simulink model "rlMpptModel"  (R2022a)
settings: Solver=ode23tb  StartTime=0.0  StopTime=0.5  FixedStep=Ts  RelTol=1e-4
model workspace (MAT data in the model file):
  Ir1 = 900
  Ir2 = 300
  Ir3 = 250
  PMmpStc = 1005
  Pmmtstc = 1004.715
  T1 = 25
  T2 = 25
  T3 = 25
  initialDuty = 0.5
libraries: spsDiodeLib x4, simulink x4, spsSeriesRLCBranchLib x4, spsPVArrayLib x3, spsCurrentMeasurementLib x1, spsIGBTDiodeLib x1, spsPWMGeneratorDCDCLib x1, spsVoltageMeasurementLib x1, rllib x1, spspowerguiLib x1
settings Model: SimulationMode=accelerator  Creator=MathWorks  LastModifiedBy=archi
settings SolverCC: AlgebraicLoopSolver=LineSearch  SolverResetMethod=Robust
settings DataIOCC: LimitDataPoints=on  SaveFormat=Array  SignalLoggingSaveFormat=ModelDataLogs
settings OptimizationCC: ExpressionDepthLimit=2147483647  LifeSpan=inf
settings DebuggingCC: UnderspecifiedInitializationDetection=Classic  MergeDetectMultiDrivingBlocksExec=none  SolverPrmCheckMsg=warning  UnconnectedInputMsg=warning  UnconnectedOutputMsg=warning  UnconnectedLineMsg=warning  AllowSymbolicDim=off  StateNameClashWarn=warning  SFUnexpectedBacktrackingDiag=warning  SFNoUnconditionalDefaultTransitionDiag=warning  SFExecutionAtInitializationDiag=none  SFMachineParentedDataDiag=warning  ArithmeticOperatorsInVariantConditions=warning
settings HardwareCC: ProdBitPerPointer=32  ProdBitPerSizeT=32  ProdBitPerPtrDiffT=32  ProdLargestAtomicFloat=None  ProdIntDivRoundTo=Undefined  ProdEndianess=Unspecified  ProdWordSize=32  ProdHWDeviceType=32-bit Generic
settings ModelReferenceCC: PropagateSignalLabelsOutOfModel=off
settings SFSimCC: SimUseLocalCustomCode=off  CustomCodeUndefinedFunction=UseInterfaceOnly
settings RTWCC: RTWUseLocalCustomCode=off
settings CodeAppCC: StateflowObjectComments=on
settings GRTTargetCC: TargetLangStandard=C89/C90 (ANSI)  CombineOutputUpdateFcns=off  GRTInterface=on
settings ConfigComp: CovMetricSettings=dw  CovSaveCumulativeToWorkspaceVar=on  CovSaveSingleToWorkspaceVar=on  CovExternalEMLEnable=off  CovSFcnEnable=off
settings SimscapeCC: SimscapeNormalizeSystem=off

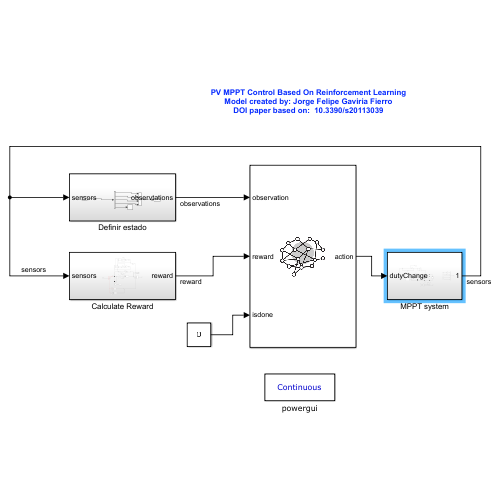
[thumbnail: Simulink's stored preview of the top-level diagram]
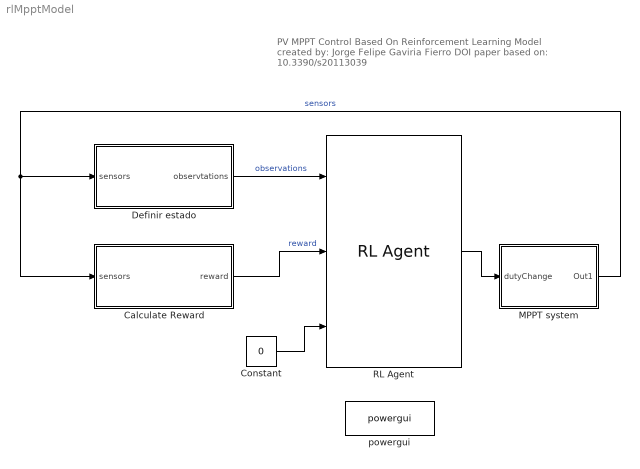
== system rlMpptModel ==
  note: PV MPPT Control Based On Reinforcement Learning
      | Model created by: Jorge Felipe Gaviria Fierro
      | DOI paper based on: 10.3390/s20113039
  Calculate Reward : Subsystem
  Constant : Constant  Value=0
  Definir estado : Subsystem
  MPPT system : Subsystem
  RL Agent : rllib/RL Agent  Agent=agentObj  ExternalActionAsInput=off  ProvideLastAction=off  ProvideCumRwd=off  TreatAsDirectFeedthrough=on  UseStrictObservationDataTypes=off
  powergui : spspowerguiLib/powergui  Priority=1  SimulationMode=Continuous  SampleTime=0.00001  frequency=60  Iterations=50  frequencyindice=0  Pbase=100e6  ErrMax=1e-4  UnitsV=kV  UnitsW=MW  buscounter=0  FunctionMessages=off  echomessages=off  EnableUseOfTLC=off  CurrentSourceSwitches=on  DisableSnubberDevices=on  DisableRonSwitches=off  DisableVfSwitches=off  DisplayEquations=off  AutomaticDiscreteSolvers=off  SolverType=Tustin/Backward Euler (TBE)  Interpol=off  ExternalGateDelay=off  methode=off  Ts=0  x0status=blocks  SPID=off  SwTol=0  HookPort=off  NonlinearTolerance=1e-4  nMaxIteration=100  ContinueOnMaxIteration=off  RestoreLinks=warning  ResistiveCurrentMeasurement=off  Frange=[0:2:500]  Ylog=off  Xlog=on  ShowGrid=off  save=off  variable=ZData  structure=0  ZoomFFT=on  StartTime=0.0  cycles=1  DisplayStyle=1  fundamental=60  FreqAxis=off  MaxFrequency=1000  frequencyindicesteady=1  RmsSteady=1  display=off
  wires:
  RL Agent/1 -> MPPT system/1(dutyChange)
  MPPT system/1(Out1) -> Calculate Reward/1(sensors), Definir estado/1(sensors)  "sensors"
  Definir estado/1(observtations) -> RL Agent/1  "observations"
  Constant/1 -> RL Agent/3
  Calculate Reward/1(reward) -> RL Agent/2  "reward"

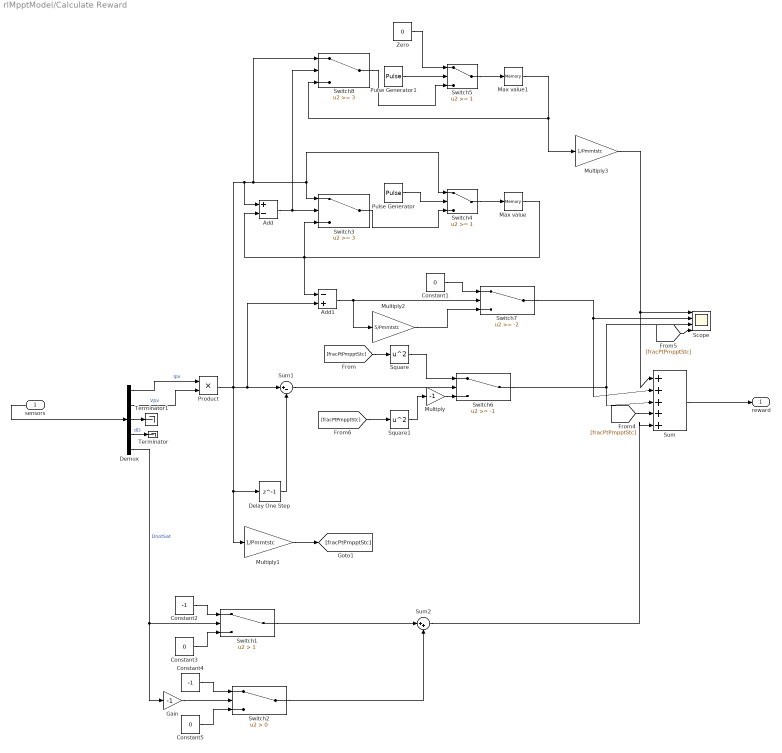
== system rlMpptModel/Calculate Reward ==
  sensors : Inport
  Add : Sum  Inputs=+-
  Add1 : Sum  Inputs=-+
  Constant1 : Constant  Value=0
  Constant2 : Constant  Value=-1
  Constant3 : Constant  Value=0
  Constant4 : Constant  Value=-1
  Constant5 : Constant  Value=0
  Delay One Step : Delay  DelayLength=1  SampleTime=0.01
  Demux : Demux  Outputs=5
  Gain : Gain  Gain=-1
  Max value : Memory
  Max value1 : Memory
  Multiply : Gain  Gain=-1
  Multiply1 : Gain  Gain=1/Pmmtstc
  Multiply2 : Gain  Gain=5/Pmmtstc
  Multiply3 : Gain  Gain=1/Pmmtstc
  Product : Product
  Pulse Generator : DiscretePulseGenerator  PulseType=Time based  Period=0.504
  Pulse Generator1 : DiscretePulseGenerator  PulseType=Time based  Period=0.0105
  Scope : Scope  NumInputPorts=4
  Square : Math  Operator=square
  Square1 : Math  Operator=square
  Sum : Sum  Inputs=|+++++
  Sum1 : Sum  Inputs=|+-
  Sum2 : Sum  Inputs=|++
  Switch1 : Switch  Criteria=u2 > Threshold  Threshold=1  SaturateOnIntegerOverflow=off  InputSameDT=off
  Switch2 : Switch  Criteria=u2 > Threshold  SaturateOnIntegerOverflow=off  InputSameDT=off
  Switch3 : Switch  Threshold=3  SaturateOnIntegerOverflow=off  InputSameDT=off
  Switch4 : Switch  Threshold=1  SaturateOnIntegerOverflow=off  InputSameDT=off
  Switch5 : Switch  Threshold=1  SaturateOnIntegerOverflow=off  InputSameDT=off
  Switch6 : Switch  Threshold=-1  SaturateOnIntegerOverflow=off  InputSameDT=off
  Switch7 : Switch  Threshold=-2  SaturateOnIntegerOverflow=off  InputSameDT=off
  Switch8 : Switch  Threshold=3  SaturateOnIntegerOverflow=off  InputSameDT=off
  Terminator : Terminator
  Terminator1 : Terminator
  Zero : Constant  Value=0  OutDataTypeStr=Inherit: Inherit via back propagation
  reward : Outport
  wires:
  sensors/1 -> Demux/1
  Demux/1 -> Product/1  "Ipv"
  Demux/2 -> Product/2  "Vpv"
  Sum/1 -> reward/1
  Delay One Step/1 -> Sum1/2
  Constant2/1 -> Switch1/1
  Constant3/1 -> Switch1/3
  Switch1/1 -> Sum2/1
  Constant5/1 -> Switch2/3
  Constant4/1 -> Switch2/1
  Gain/1 -> Switch2/2
  Switch2/1 -> Sum2/2
  Demux/4 -> Terminator/1  "dD"
  Demux/3 -> Terminator1/1
  Sum2/1 -> Sum/5
  Demux/5 -> Switch1/2, Gain/1  "DnotSat"
  Max value/1 -> Add1/1, Switch3/3, Add/2
  Pulse Generator/1 -> Switch4/2
  Product/1 -> Multiply1/1, Delay One Step/1, Sum1/1, Add1/2, Add/1, Switch8/1, Switch3/1, Switch4/1
  Switch4/1 -> Max value/1
  Switch7/1 -> Sum/2, Scope/2
  Add/1 -> Switch8/2, Switch3/2
  Sum1/1 -> Switch6/2
  Square/1 -> Switch6/1
  Square1/1 -> Multiply/1
  Switch6/1 -> Sum/3, Scope/3
  Multiply3/1 -> Scope/1, Sum/1
  Add1/1 -> Multiply2/1, Switch7/2
  Constant1/1 -> Switch7/1
  Switch5/1 -> Max value1/1
  Switch3/1 -> Switch4/3
  Pulse Generator1/1 -> Switch5/2
  Max value1/1 -> Multiply3/1, Switch8/3
  Switch8/1 -> Switch5/3
  Zero/1 -> Switch5/1
  Multiply1/1 -> [fracPtPmpptStc]
  [fracPtPmpptStc] -> Square/1
  [fracPtPmpptStc] -> Sum/4
  [fracPtPmpptStc] -> Scope/4
  [fracPtPmpptStc] -> Square1/1
  Multiply2/1 -> Switch7/3
  Multiply/1 -> Switch6/3

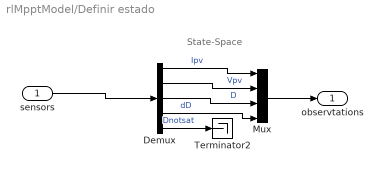
== system rlMpptModel/Definir estado ==
  note: State-Space
  sensors : Inport
  Demux : Demux  Outputs=5
  Mux : Mux
  Terminator2 : Terminator
  observtations : Outport
  wires:
  Demux/4 -> Mux/4  "dD"
  Demux/1 -> Mux/1  "Ipv"
  Demux/2 -> Mux/2  "Vpv"
  sensors/1 -> Demux/1
  Mux/1 -> observtations/1
  Demux/3 -> Mux/3  "D"
  Demux/5 -> Terminator2/1  "Dnotsat"

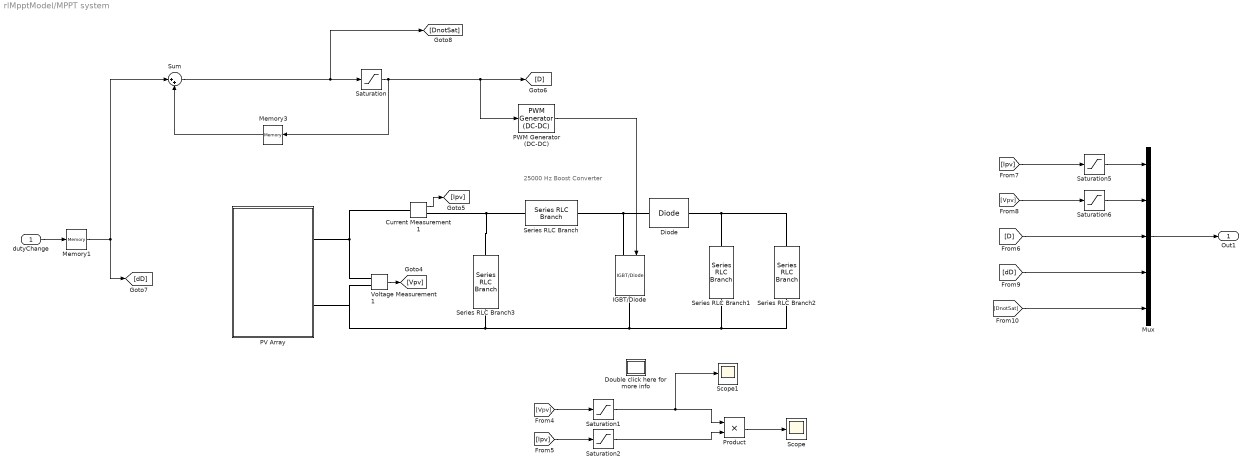
== system rlMpptModel/MPPT system ==
  note: 25000 Hz
      | Boost Converter
  dutyChange : Inport
  Current Measurement1 : spsCurrentMeasurementLib/Current Measurement  PhasorSimulation=off  OutputType=Complex  PSBequivalent=0
  Diode : spsDiodeLib/Diode  Ron=0.001  Lon=0  Vf=0.8  IC=0  UseSnubber=0  Rs=500  Cs=inf  Measurements=off
  Double click here for more info : Subsystem
      settings: OpenFcn=showdemo(bdroot(gcb))
      mask Display: disp('?')
  IGBT/Diode : spsIGBTDiodeLib/IGBT//Diode  Ron=1e-3  Rs=1e5  Cs=inf  Measurements=off
  Memory1 : Memory  InheritSampleTime=on
  Memory3 : Memory  InitialCondition=initialDuty  InheritSampleTime=on
  Mux : Mux  Inputs=5
  PV Array : Subsystem
  PWM Generator (DC-DC) : spsPWMGeneratorDCDCLib/PWM Generator (DC-DC)  Fsw=25000  Ts=0
  Product : Product
  Saturation : Saturate  UpperLimit=1  LowerLimit=0
  Saturation1 : Saturate  UpperLimit=1000000000000000  LowerLimit=0
  Saturation2 : Saturate  UpperLimit=1000000000000000000  LowerLimit=0
  Saturation5 : Saturate  UpperLimit=1000000000000  LowerLimit=0
  Saturation6 : Saturate  UpperLimit=10000000000000000  LowerLimit=0
  Scope : Scope
  Scope1 : Scope
  Series RLC Branch : spsSeriesRLCBranchLib/Series RLC Branch  LConnTagsString=__new0  RConnTagsString=__new0  BranchType=L  Resistance=1  Inductance=2.057e-3  SetiL0=off  InitialCurrent=0  Capacitance=1e-6  Setx0=off  InitialVoltage=0  Measurements=None
  Series RLC Branch1 : spsSeriesRLCBranchLib/Series RLC Branch  LConnTagsString=__new0  RConnTagsString=__new0  BranchType=C  Resistance=1  Inductance=1e-3  SetiL0=off  InitialCurrent=0  Capacitance=1.29e-05  Setx0=off  InitialVoltage=0  Measurements=None
  Series RLC Branch2 : spsSeriesRLCBranchLib/Series RLC Branch  LConnTagsString=__new0  RConnTagsString=__new0  BranchType=R  Resistance=61.71003717  Inductance=1e-3  SetiL0=off  InitialCurrent=0  Capacitance=1e-6  Setx0=off  InitialVoltage=0  Measurements=None
  Series RLC Branch3 : spsSeriesRLCBranchLib/Series RLC Branch  LConnTagsString=__new0  RConnTagsString=__new0  BranchType=C  Resistance=1e-4  Inductance=1.032e-3  SetiL0=off  InitialCurrent=0  Capacitance=3e-3  Setx0=off  InitialVoltage=0  Measurements=None
  Sum : Sum  Inputs=|++
  Voltage Measurement1 : spsVoltageMeasurementLib/Voltage Measurement  PhasorSimulation=off  OutputType=Complex  PSBequivalent=0
  Out1 : Outport
  wires:
  dutyChange/1 -> Memory1/1
  [Vpv] -> Saturation1/1
  Current Measurement1/1 -> [Ipv]
  [Ipv] -> Saturation2/1
  Voltage Measurement1/1 -> [Vpv]
  Mux/1 -> Out1/1
  PWM Generator (DC-DC)/1 -> IGBT/Diode/1
  [DnotSat] -> Mux/5
  [dD] -> Mux/4
  [D] -> Mux/3
  Memory1/1 -> Sum/1, [dD]
  Memory3/1 -> Sum/2
  Saturation1/1 -> Scope1/1, Product/1
  Saturation2/1 -> Product/2
  [Ipv] -> Saturation5/1
  [Vpv] -> Saturation6/1
  Saturation5/1 -> Mux/1
  Saturation6/1 -> Mux/2
  Sum/1 -> [DnotSat], Saturation/1
  Saturation/1 -> PWM Generator (DC-DC)/1, [D], Memory3/1
  Product/1 -> Scope/1
  connections:
  Series RLC Branch2/RConn1 -- Series RLC Branch1/RConn1 -- Voltage Measurement1/LConn2 -- PV Array/RConn2 -- Series RLC Branch3/RConn1 -- IGBT/Diode/RConn1
  Series RLC Branch3/LConn1 -- Current Measurement1/RConn1 -- Series RLC Branch/LConn1
  PV Array/RConn1 -- Voltage Measurement1/LConn1 -- Current Measurement1/LConn1
  Diode/RConn1 -- Series RLC Branch1/LConn1 -- Series RLC Branch2/LConn1
  Diode/LConn1 -- IGBT/Diode/LConn1 -- Series RLC Branch/RConn1

== system rlMpptModel/MPPT system/Double click here for more info ==

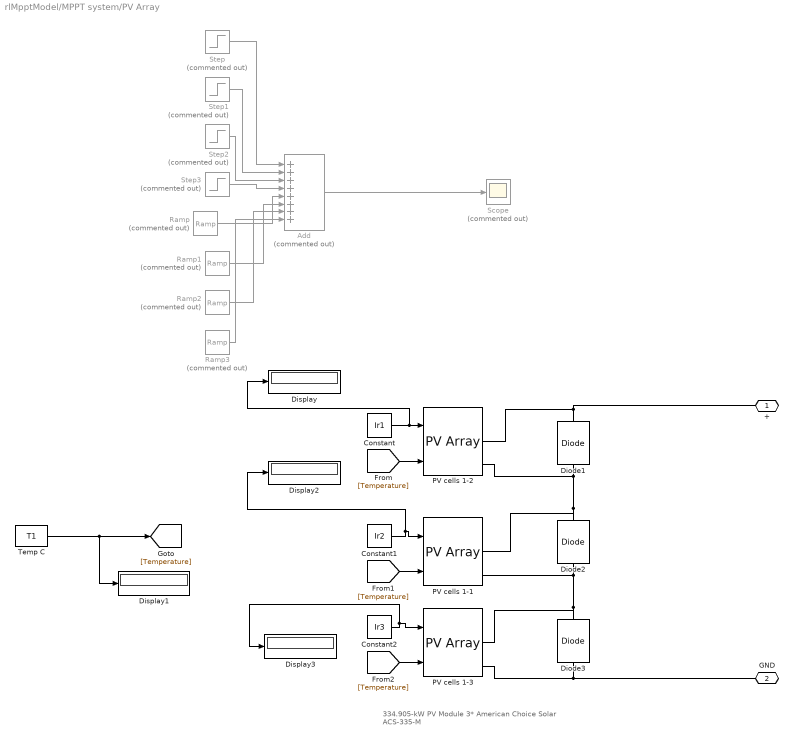
== system rlMpptModel/MPPT system/PV Array ==
  note: 334.905-kW  PV Module
      | 3* American Choice Solar ACS-335-M
  Add : Sum  Commented=on  Inputs=++++++++
  Constant : Constant  Value=Ir1
  Constant1 : Constant  Value=Ir2
  Constant2 : Constant  Value=Ir3
  Diode1 : spsDiodeLib/Diode  Ron=0.001  Lon=0  Vf=0.7  IC=0  UseSnubber=off  Rs=1e5*inf  Cs=inf  Measurements=off
  Diode2 : spsDiodeLib/Diode  Ron=0.001  Lon=0  Vf=0.7  IC=0  UseSnubber=off  Rs=1e5*inf  Cs=inf  Measurements=off
  Diode3 : spsDiodeLib/Diode  Ron=0.001  Lon=0  Vf=0.7  IC=0  UseSnubber=off  Rs=1e5*inf  Cs=inf  Measurements=off
  Display{,1..3} (4 alike) : Display
  PV cells 1-1 : spsPVArrayLib/PV Array  Npar=1  Nser=1  PlotType=array @ 25 deg.C & specified irradiances  S_vec="[ 1000  500  100 ]"  Temp_C_vec="[ 45 25  ]"  ModuleName=User-defined  PlotWhenSelected=off  Pm=334.905  Ncell=80  Voc=49.9  Isc=9  Vm=41.5  Im=8.07  beta_Voc_pc=-0.36  alpha_Isc_pc=0.09  beta_Voc=-0.17964  alpha_Isc=0.0081  IL=9.0297  I0=3.1312e-10  nI=1.0111  Rsh=77.6407  Rs=0.25633  RobustModel=off  RobustCellTemperature=25  BAL=on  Tc=1e-5  Tfilter=5e-5
  PV cells 1-2 : spsPVArrayLib/PV Array  Npar=1  Nser=1  PlotType=array @ 1000 W/m2 & specified temperatures  S_vec="[ 1000  500  100 ]"  Temp_C_vec=[ 20 ]  ModuleName=User-defined  PlotWhenSelected=off  Pm=334.905  Ncell=80  Voc=49.9  Isc=9  Vm=41.5  Im=8.07  beta_Voc_pc=-0.36  alpha_Isc_pc=0.09  beta_Voc=-0.17964  alpha_Isc=0.0081  IL=9.0297  I0=3.1312e-10  nI=1.0111  Rsh=77.6407  Rs=0.25633  RobustModel=off  RobustCellTemperature=25  BAL=on  Tc=1e-5  Tfilter=5e-5
  PV cells 1-3 : spsPVArrayLib/PV Array  Npar=1  Nser=1  PlotType=array @ 25 deg.C & specified irradiances  S_vec="[ 1000  500  100 ]"  Temp_C_vec="[ 45 25  ]"  ModuleName=User-defined  PlotWhenSelected=off  Pm=334.905  Ncell=80  Voc=49.9  Isc=9  Vm=41.5  Im=8.07  beta_Voc_pc=-0.36  alpha_Isc_pc=0.09  beta_Voc=-0.17964  alpha_Isc=0.0081  IL=9.0297  I0=3.1312e-10  nI=1.0111  Rsh=77.6407  Rs=0.25633  RobustModel=off  RobustCellTemperature=25  BAL=on  Tc=1e-5  Tfilter=5e-5
  Ramp : simulink/Sources/Ramp  Commented=on  slope=100  start=2.3  InitialOutput=0
  Ramp1 : simulink/Sources/Ramp  Commented=on  slope=-100  start=4  InitialOutput=0
  Ramp2 : simulink/Sources/Ramp  Commented=on  slope=-100  start=5  InitialOutput=0
  Ramp3 : simulink/Sources/Ramp  Commented=on  slope=100  start=7  InitialOutput=0
  Scope : Scope  Commented=on
  Step : Step  Commented=on  Time=0  After=1000  SampleTime=0
  Step1 : Step  Commented=on  Time=0.6  After=-230  SampleTime=0
  Step2 : Step  Commented=on  After=-200  SampleTime=0
  Step3 : Step  Commented=on  Time=1.5  After=-200  SampleTime=0
  Temp C : Constant  Value=T1
  + : PMIOPort  Side=Right
  GND : PMIOPort  Port=2  Side=Right
  wires:
  Temp C/1 -> [Temperature], Display1/1
  Step/1 -> Add/1
  Step1/1 -> Add/2
  Step2/1 -> Add/3
  Step3/1 -> Add/4
  Ramp/1 -> Add/5
  Ramp1/1 -> Add/6
  Ramp2/1 -> Add/7
  Ramp3/1 -> Add/8
  Add/1 -> Scope/1
  Constant1/1 -> PV cells 1-1/1, Display2/1
  Constant2/1 -> PV cells 1-3/1, Display3/1
  Constant/1 -> PV cells 1-2/1, Display/1
  [Temperature] -> PV cells 1-2/2
  [Temperature] -> PV cells 1-1/2
  [Temperature] -> PV cells 1-3/2
  connections:
  PV cells 1-1/RConn1 -- Diode2/RConn1 -- PV cells 1-2/RConn2 -- Diode1/LConn1
  PV cells 1-2/RConn1 -- +/RConn1 -- Diode1/RConn1
  Diode2/LConn1 -- PV cells 1-3/RConn1 -- Diode3/RConn1 -- PV cells 1-1/RConn2
  PV cells 1-3/RConn2 -- GND/RConn1 -- Diode3/LConn1
